simulink model "MyHistogramEqualizationForHDLCoder"  (R2024b)
settings: Solver=VariableStepAuto  StartTime=0.0  StopTime=10.0  RelTol=1e-3
libraries: visionhdlio x6, visionsources x1
settings Model: Creator=snmz4  LastModifiedBy=snmz4

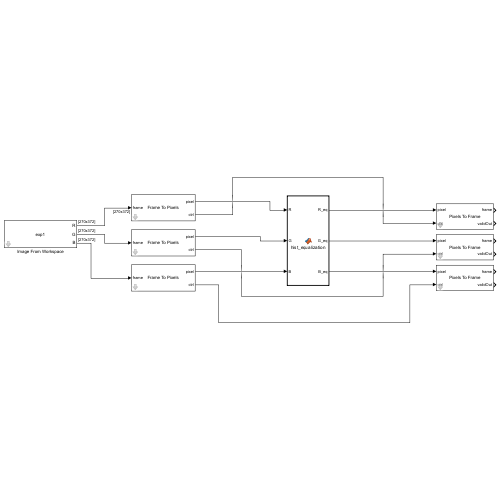
[thumbnail: Simulink's stored preview of the top-level diagram]
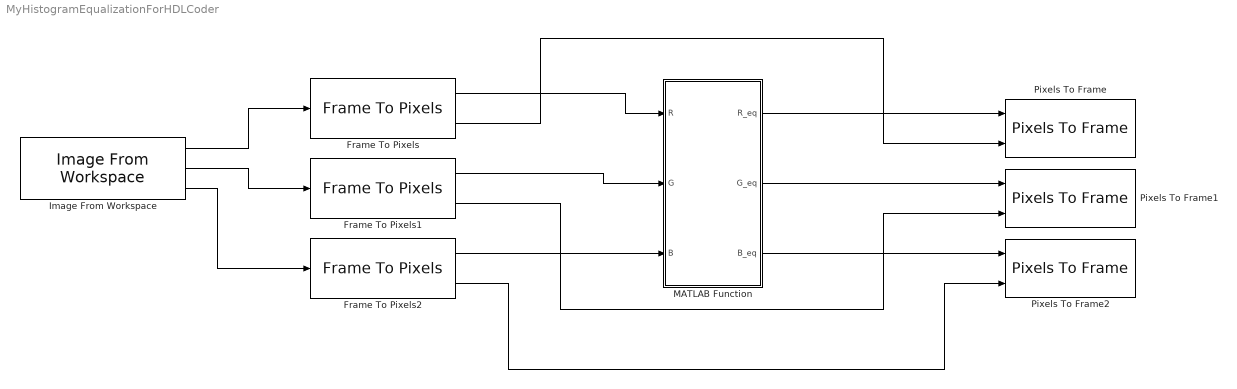
== system MyHistogramEqualizationForHDLCoder ==
  Frame To Pixels : visionhdlio/Frame To Pixels  NumComponents=1  NumPixels=1  VideoFormat=Custom  ActivePixelsPerLine=32  ActiveVideoLines=18  TotalPixelsPerLine=42  TotalVideoLines=28  StartingActiveLine=6  FrontPorch=5  SampleTime=0  VideoFormatCache=Custom  ActivePixelsPerLineCache=32  ActiveVideoLinesCache=18  TotalPixelsPerLineCache=42  TotalVideoLinesCache=28  StartingActiveLineCache=6  FrontPorchCache=5
  Frame To Pixels1 : visionhdlio/Frame To Pixels  NumComponents=1  NumPixels=1  VideoFormat=Custom  ActivePixelsPerLine=32  ActiveVideoLines=18  TotalPixelsPerLine=42  TotalVideoLines=28  StartingActiveLine=6  FrontPorch=5  SampleTime=0  VideoFormatCache=Custom  ActivePixelsPerLineCache=32  ActiveVideoLinesCache=18  TotalPixelsPerLineCache=42  TotalVideoLinesCache=28  StartingActiveLineCache=6  FrontPorchCache=5
  Frame To Pixels2 : visionhdlio/Frame To Pixels  NumComponents=1  NumPixels=1  VideoFormat=Custom  ActivePixelsPerLine=32  ActiveVideoLines=18  TotalPixelsPerLine=42  TotalVideoLines=28  StartingActiveLine=6  FrontPorch=5  SampleTime=0  VideoFormatCache=Custom  ActivePixelsPerLineCache=32  ActiveVideoLinesCache=18  TotalPixelsPerLineCache=42  TotalVideoLinesCache=28  StartingActiveLineCache=6  FrontPorchCache=5
  Image From Workspace : visionsources/Image From Workspace  Tag=vipblks_nd  ImageValue=exp1  Ts=inf  imagePorts=Separate color signals  OutPortLabels=R|G|B  ImageDataType=Fixed-point  Signed=on  WordLength=16  sdImageDataType=sfix(16)  FractionLengthMode=User-defined  FractionLength=15
  MATLAB Function : MATLAB Function  TreatAsAtomicUnit=on
  Pixels To Frame : visionhdlio/Pixels To Frame  NumComponents=1  NumPixels=1  VideoFormat=1080p  ActivePixelsPerLine=1920  ActiveVideoLines=1080  TotalPixelsPerLine=2200  TotalVideoLines=1125  VideoFormatCache=1080p  ActivePixelsPerLineCache=32  ActiveVideoLinesCache=18  TotalPixelsPerLineCache=42  TotalVideoLinesCache=28
  Pixels To Frame1 : visionhdlio/Pixels To Frame  NumComponents=1  NumPixels=1  VideoFormat=1080p  ActivePixelsPerLine=1920  ActiveVideoLines=1080  TotalPixelsPerLine=2200  TotalVideoLines=1125  VideoFormatCache=1080p  ActivePixelsPerLineCache=32  ActiveVideoLinesCache=18  TotalPixelsPerLineCache=42  TotalVideoLinesCache=28
  Pixels To Frame2 : visionhdlio/Pixels To Frame  NumComponents=1  NumPixels=1  VideoFormat=1080p  ActivePixelsPerLine=1920  ActiveVideoLines=1080  TotalPixelsPerLine=2200  TotalVideoLines=1125  VideoFormatCache=1080p  ActivePixelsPerLineCache=32  ActiveVideoLinesCache=18  TotalPixelsPerLineCache=42  TotalVideoLinesCache=28
  wires:
  Frame To Pixels/1 -> MATLAB Function/1(R)
  Image From Workspace/1 -> Frame To Pixels/1
  Image From Workspace/2 -> Frame To Pixels1/1
  Image From Workspace/3 -> Frame To Pixels2/1
  Frame To Pixels1/1 -> MATLAB Function/2(G)
  Frame To Pixels2/1 -> MATLAB Function/3(B)
  MATLAB Function/2(G_eq) -> Pixels To Frame1/1
  MATLAB Function/1(R_eq) -> Pixels To Frame/1
  MATLAB Function/3(B_eq) -> Pixels To Frame2/1
  Frame To Pixels/2 -> Pixels To Frame/2
  Frame To Pixels1/2 -> Pixels To Frame1/2
  Frame To Pixels2/2 -> Pixels To Frame2/2

== matlab function MyHistogramEqualizationForHDLCoder/MATLAB Function ==
  data: R input; R_eq output; G input; B input; G_eq output; B_eq output
function [R_eq, G_eq, B_eq] = hist_equalization(R, G, B)
%#codegen
% Histogram Equalization işlemini LUT (Lookup Table) kullanarak gerçekleştirir.
% Bu örnekte LUT, basitçe 0'dan 255'e kadar olan değerlerden oluşan bir identity mapping'tir.
% Gerçek uygulamada, LUT değerlerini görüntünün histogram eşitleme sonucuna göre 
% offline olarak hesaplayıp sabit (coder.const) olarak tanımlamanız gerekir.
%
% Giriş:
%   R, G, B  : uint8 formatında piksel değerleri
%   ctrl     : Frame bilgisi gibi kontrol sinyali (HDL akışında korunması gereken)
%
% Çıkış:
%   R_eq, G_eq, B_eq : Histogram eşitleme sonrası çıkış piksel değerleri
%   ctrl_out         : Girişte gelen ctrl sinyali, değişiklik olmadan aktarılır

% LUT sabit tanımlama (placeholder - identity mapping)
lut = coder.const(uint8(0:255));

% LUT kullanarak eşitleme: uint8 değerlerin 0-255 aralığında olduğunu varsayarız.
R_eq = lut(uint8(R) + 1); % MATLAB'da indeks 1'den başladığı için +1 eklenir.
G_eq = lut(uint8(G) + 1);
B_eq = lut(uint8(B) + 1);

% Eğer ctrl bir bus sinyaliyse, bunu uygun şekilde kopyala
%if isa(ctrl, 'bus')  % Eğer bus sinyali ise
 %   ctrl_out = ctrl;  % Bus sinyalini koru
%else
    % Eğer bus değilse, uygun şekilde bir bus nesnesi oluştur
 %   ctrl_out = Simulink.Bus.createMATLABStruct('ctrlBus');
  %  ctrl_out.signal = ctrl; % Sinyali atama
%end
